simulink model "rocket_sim"  (R2023a)
settings: Solver=VariableStepAuto  StartTime=0.0  StopTime=480  RelTol=1e-3
undefined symbols (not defined in the file or in its folder): Earth, WGS84
libraries: simulink x55, slpidlib x10, aerolibconvert2 x7, matrix_library x4, aerolibasang x3, aerolibtransform2 x2, aerolibatmos2 x2, shared6dof x1, sharedtransform x1
(part 3 of 3)

== system rocket_sim/栅格舵控制器/栅格舵/F01 ==
  Th : Inport
  F : Inport  Port=2
  Constant : Constant  Value=0
  Saturation : Saturate  UpperLimit=1  LowerLimit=0
  Step1 : Step  Time=200  SampleTime=0
  Step2 : Step  Time=480  SampleTime=0
  Switch2 : Switch  Criteria=u2 > Threshold  SaturateOnIntegerOverflow=off  InputSameDT=off
  Switch3 : Switch  Criteria=u2 > Threshold  SaturateOnIntegerOverflow=off  InputSameDT=off
  Switch4 : Switch  Criteria=u2 > Threshold  SaturateOnIntegerOverflow=off  InputSameDT=off
  故障 : Subsystem
  退化 : Subsystem
  Out1 : Outport
  wires:
  Step1/1 -> Switch4/3
  退化/1(Out1) -> Switch3/3, Switch2/1
  F/1 -> Switch4/2
  Switch3/1 -> Switch2/3
  故障/1(Out1) -> Switch3/1
  Step2/1 -> Switch2/2
  Switch4/1 -> Switch3/2
  Th/1 -> 故障/1(Th), 退化/1(Th)
  Constant/1 -> Switch4/1
  Switch2/1 -> Saturation/1
  Saturation/1 -> Out1/1

== system rocket_sim/栅格舵控制器/栅格舵/F02 ==
  F : Inport
  Constant1 : Constant  Value=0
  Gain : Gain  Gain=0
  Gain1 : Gain
  Step : Step  Time=0  SampleTime=0
  Step1 : Step  Time=100  SampleTime=0
  Step2 : Step  Time=200  SampleTime=0
  Switch2 : Switch  Criteria=u2 > Threshold  SaturateOnIntegerOverflow=off  InputSameDT=off
  Switch4 : Switch  Criteria=u2 > Threshold  SaturateOnIntegerOverflow=off  InputSameDT=off
  Switch5 : Switch  Criteria=u2 > Threshold  SaturateOnIntegerOverflow=off  InputSameDT=off
  out2 : Outport
  wires:
  Switch5/1 -> Switch4/2
  Switch4/1 -> Switch2/3
  Constant1/1 -> Switch5/1
  Step1/1 -> Switch5/3
  Gain/1 -> Switch4/1
  Step2/1 -> Switch2/2
  Gain1/1 -> Switch4/3, Switch2/1
  Switch2/1 -> out2/1
  Step/1 -> Gain/1, Gain1/1
  F/1 -> Switch5/2

== system rocket_sim/栅格舵控制器/栅格舵/F03 ==
  Th : Inport
  F : Inport  Port=2
  Constant : Constant  Value=0
  Saturation : Saturate  UpperLimit=1  LowerLimit=0
  Step1 : Step  Time=200  SampleTime=0
  Step2 : Step  Time=480  SampleTime=0
  Switch2 : Switch  Criteria=u2 > Threshold  SaturateOnIntegerOverflow=off  InputSameDT=off
  Switch3 : Switch  Criteria=u2 > Threshold  SaturateOnIntegerOverflow=off  InputSameDT=off
  Switch4 : Switch  Criteria=u2 > Threshold  SaturateOnIntegerOverflow=off  InputSameDT=off
  故障 : Subsystem
  退化 : Subsystem
  Out1 : Outport
  wires:
  Step1/1 -> Switch4/3
  退化/1(Out1) -> Switch3/3, Switch2/1
  F/1 -> Switch4/2
  Switch3/1 -> Switch2/3
  故障/1(Out1) -> Switch3/1
  Step2/1 -> Switch2/2
  Switch4/1 -> Switch3/2
  Th/1 -> 故障/1(Th), 退化/1(Th)
  Switch2/1 -> Saturation/1
  Saturation/1 -> Out1/1
  Constant/1 -> Switch4/1

== system rocket_sim/栅格舵控制器/栅格舵/F04 ==
  F : Inport
  Constant1 : Constant  Value=0
  Gain : Gain  Gain=0
  Gain1 : Gain
  Step : Step  Time=0  SampleTime=0
  Step1 : Step  Time=100  SampleTime=0
  Step2 : Step  Time=200  SampleTime=0
  Switch2 : Switch  Criteria=u2 > Threshold  SaturateOnIntegerOverflow=off  InputSameDT=off
  Switch4 : Switch  Criteria=u2 > Threshold  SaturateOnIntegerOverflow=off  InputSameDT=off
  Switch5 : Switch  Criteria=u2 > Threshold  SaturateOnIntegerOverflow=off  InputSameDT=off
  out2 : Outport
  wires:
  Switch5/1 -> Switch4/2
  Switch4/1 -> Switch2/3
  Constant1/1 -> Switch5/1
  Step1/1 -> Switch5/3
  Gain/1 -> Switch4/1
  Step2/1 -> Switch2/2
  Gain1/1 -> Switch4/3, Switch2/1
  Switch2/1 -> out2/1
  Step/1 -> Gain/1, Gain1/1
  F/1 -> Switch5/2

== system rocket_sim/动力系统模块/喷管/F01/故障 ==
  Th : Inport
  Band-Limited White Noise1 : simulink/Sources/Band-Limited White Noise  Cov=[0.1]  Ts=0.1  seed=[23341]
  Clock1 : Clock
  Gain : Gain  Gain=0.9
  Gain2 : Gain  Gain=0.001
  Gain3 : Gain  Gain=-2.1950e-06
  Integrator1 : Integrator
  Math Function1 : Math
  Saturation : Saturate  UpperLimit=0.9  LowerLimit=0.5
  Sum2 : Sum  Inputs=|++
  Sum3 : Sum  Inputs=|++
  Out1 : Outport
  wires:
  Gain2/1 -> Sum2/2
  Th/1 -> Sum3/2
  Band-Limited White Noise1/1 -> Integrator1/1
  Clock1/1 -> Sum3/1
  Integrator1/1 -> Gain2/1
  Sum3/1 -> Gain3/1
  Gain3/1 -> Math Function1/1
  Saturation/1 -> Out1/1
  Sum2/1 -> Saturation/1
  Math Function1/1 -> Gain/1
  Gain/1 -> Sum2/1

== system rocket_sim/动力系统模块/喷管/F01/退化 ==
  Th : Inport
  Band-Limited White Noise1 : simulink/Sources/Band-Limited White Noise  Cov=[0.1]  Ts=0.1  seed=[23341]
  Clock1 : Clock
  Gain2 : Gain  Gain=0.0001
  Gain3 : Gain  Gain=-2.1950e-05
  Integrator1 : Integrator
  Math Function1 : Math
  Saturation : Saturate  UpperLimit=1  LowerLimit=0.5
  Scope : Scope
  Sum2 : Sum  Inputs=|++
  Sum3 : Sum  Inputs=|++
  Out1 : Outport
  wires:
  Gain2/1 -> Sum2/2
  Th/1 -> Sum3/2
  Band-Limited White Noise1/1 -> Integrator1/1
  Clock1/1 -> Sum3/1
  Integrator1/1 -> Gain2/1
  Sum3/1 -> Gain3/1
  Math Function1/1 -> Sum2/1
  Gain3/1 -> Math Function1/1
  Saturation/1 -> Out1/1
  Sum2/1 -> Scope/1, Saturation/1

== system rocket_sim/动力系统模块/氧涡轮/F01/故障 ==
  Th : Inport
  Band-Limited White Noise : simulink/Sources/Band-Limited White Noise  Cov=[0.1]  Ts=1  seed=[23341]
  Clock1 : Clock
  Gain : Gain  Gain=-4.65e-6
  Gain1 : Gain  Gain=0.8
  Integrator : Integrator
  Math Function : Math
  Saturation : Saturate  UpperLimit=1  LowerLimit=0.5
  Sum : Sum  Inputs=|++
  Sum1 : Sum  Inputs=|++
  σ : Gain  Gain=1e-3
  Out1 : Outport
  wires:
  Band-Limited White Noise/1 -> Integrator/1
  Clock1/1 -> Sum/1
  Integrator/1 -> σ/1
  Gain/1 -> Math Function/1
  σ/1 -> Sum1/2
  Sum/1 -> Gain/1
  Sum1/1 -> Saturation/1
  Saturation/1 -> Out1/1
  Math Function/1 -> Gain1/1
  Gain1/1 -> Sum1/1
  Th/1 -> Sum/2

== system rocket_sim/动力系统模块/氧涡轮/F01/退化 ==
  Th : Inport
  Band-Limited White Noise : simulink/Sources/Band-Limited White Noise  Cov=[0.1]  Ts=1  seed=[23341]
  Clock1 : Clock
  Gain : Gain  Gain=-4.65e-5
  Integrator : Integrator
  Math Function : Math
  Saturation : Saturate  UpperLimit=1  LowerLimit=0.5
  Sum : Sum  Inputs=|++
  Sum1 : Sum  Inputs=|++
  σ : Gain  Gain=1e-3
  Out1 : Outport
  wires:
  Band-Limited White Noise/1 -> Integrator/1
  Th/1 -> Sum/2
  Clock1/1 -> Sum/1
  Integrator/1 -> σ/1
  Gain/1 -> Math Function/1
  Math Function/1 -> Sum1/1
  σ/1 -> Sum1/2
  Sum/1 -> Gain/1
  Sum1/1 -> Saturation/1
  Saturation/1 -> Out1/1

== system rocket_sim/动力系统模块/液氧主阀/F01/故障 ==
  Th : Inport
  Band-Limited White Noise : simulink/Sources/Band-Limited White Noise  Cov=[0.1]  Ts=0.1  seed=[23341]
  Clock2 : Clock
  Constant : Constant  Value=0.9
  Gain : Gain  Gain=-0.00012
  Gain1 : Gain  Gain=0.0001
  Integrator : Integrator
  MATLAB Function1 : MATLAB Function  TreatAsAtomicUnit=on
  Sum : Sum  Inputs=|++
  Sum1 : Sum  Inputs=|+++
  Out1 : Outport
  wires:
  Gain/1 -> Sum1/1
  Th/1 -> Sum/2
  MATLAB Function1/1(y) -> Gain/1
  Sum/1 -> MATLAB Function1/1(t)
  Constant/1 -> Sum1/2
  Clock2/1 -> Sum/1
  Sum1/1 -> Out1/1
  Gain1/1 -> Sum1/3
  Band-Limited White Noise/1 -> Integrator/1
  Integrator/1 -> Gain1/1

== system rocket_sim/动力系统模块/液氧主阀/F01/退化 ==
  Th : Inport
  Band-Limited White Noise : simulink/Sources/Band-Limited White Noise  Cov=[0.1]  Ts=0.1  seed=[23341]
  Clock2 : Clock
  Constant : Constant
  Gain : Gain  Gain=-0.0012
  Gain1 : Gain  Gain=0.0001
  Integrator : Integrator
  MATLAB Function1 : MATLAB Function  TreatAsAtomicUnit=on
  Sum : Sum  Inputs=|++
  Sum1 : Sum  Inputs=|+++
  Out1 : Outport
  wires:
  Gain/1 -> Sum1/1
  Th/1 -> Sum/2
  MATLAB Function1/1(y) -> Gain/1
  Sum/1 -> MATLAB Function1/1(t)
  Constant/1 -> Sum1/2
  Clock2/1 -> Sum/1
  Sum1/1 -> Out1/1
  Band-Limited White Noise/1 -> Integrator/1
  Integrator/1 -> Gain1/1
  Gain1/1 -> Sum1/3

== system rocket_sim/动力系统模块/液氧泵/F01/故障 ==
  Th : Inport
  Add1 : Sum  Inputs=+++
  Band-Limited White Noise1 : simulink/Sources/Band-Limited White Noise  Cov=[0.1]  Ts=1  seed=[23341]
  Clock1 : Clock
  Constant3 : Constant  Value=0.8
  Integrator1 : Integrator
  Scope : Scope
  Sum : Sum  Inputs=|++
  μ1 : Gain  Gain=-4.1667e-06
  σ1 : Gain  Gain=1e-3
  Out1 : Outport
  wires:
  Th/1 -> Sum/2
  Sum/1 -> Scope/1, μ1/1
  Clock1/1 -> Sum/1
  Band-Limited White Noise1/1 -> Integrator1/1
  Integrator1/1 -> σ1/1
  σ1/1 -> Add1/2
  μ1/1 -> Add1/3
  Constant3/1 -> Add1/1
  Add1/1 -> Out1/1

== system rocket_sim/动力系统模块/液氧泵/F01/退化 ==
  Th : Inport
  Add : Sum  Inputs=+++
  Band-Limited White Noise : simulink/Sources/Band-Limited White Noise  Cov=[0.1]  Ts=1  seed=[23341]
  Clock : Clock
  Constant2 : Constant
  Integrator : Integrator
  Sum : Sum  Inputs=|++
  μ : Gain  Gain=-6.94e-5
  σ : Gain  Gain=1e-3
  Out1 : Outport
  wires:
  Band-Limited White Noise/1 -> Integrator/1
  σ/1 -> Add/2
  Integrator/1 -> σ/1
  Constant2/1 -> Add/1
  Add/1 -> Out1/1
  μ/1 -> Add/3
  Clock/1 -> Sum/1
  Sum/1 -> μ/1
  Th/1 -> Sum/2

== system rocket_sim/动力系统模块/液氧管路/F01/故障 ==
  Th : Inport
  Add1 : Sum  Inputs=+++
  Band-Limited White Noise1 : simulink/Sources/Band-Limited White Noise  Cov=[0.1]  Ts=1  seed=[23341]
  Clock1 : Clock
  Constant3 : Constant  Value=0.8
  Integrator1 : Integrator
  Scope : Scope
  Sum : Sum  Inputs=|++
  μ1 : Gain  Gain=-2.0833e-06
  σ1 : Gain  Gain=1e-3
  Out1 : Outport
  wires:
  Th/1 -> Sum/2
  Sum/1 -> Scope/1, μ1/1
  Clock1/1 -> Sum/1
  Band-Limited White Noise1/1 -> Integrator1/1
  Integrator1/1 -> σ1/1
  σ1/1 -> Add1/2
  μ1/1 -> Add1/3
  Constant3/1 -> Add1/1
  Add1/1 -> Out1/1

== system rocket_sim/动力系统模块/液氧管路/F01/退化 ==
  Th : Inport
  Add : Sum  Inputs=+++
  Band-Limited White Noise : simulink/Sources/Band-Limited White Noise  Cov=[0.1]  Ts=1  seed=[23341]
  Clock : Clock
  Constant2 : Constant
  Integrator : Integrator
  Sum : Sum  Inputs=|++
  μ : Gain  Gain=-2.0833e-05
  σ : Gain  Gain=1e-3
  Out1 : Outport
  wires:
  Band-Limited White Noise/1 -> Integrator/1
  σ/1 -> Add/2
  Integrator/1 -> σ/1
  Constant2/1 -> Add/1
  Add/1 -> Out1/1
  μ/1 -> Add/3
  Clock/1 -> Sum/1
  Sum/1 -> μ/1
  Th/1 -> Sum/2

== system rocket_sim/动力系统模块/煤油主阀/F01/故障 ==
  Th : Inport
  Band-Limited White Noise : simulink/Sources/Band-Limited White Noise  Cov=[0.1]  Ts=0.1  seed=[23341]
  Clock2 : Clock
  Constant : Constant  Value=0.9
  Gain : Gain  Gain=-0.00012
  Gain1 : Gain  Gain=0.0001
  Integrator : Integrator
  MATLAB Function1 : MATLAB Function  TreatAsAtomicUnit=on
  Sum : Sum  Inputs=|++
  Sum1 : Sum  Inputs=|+++
  Out1 : Outport
  wires:
  Gain/1 -> Sum1/1
  Th/1 -> Sum/2
  MATLAB Function1/1(y) -> Gain/1
  Sum/1 -> MATLAB Function1/1(t)
  Constant/1 -> Sum1/2
  Clock2/1 -> Sum/1
  Sum1/1 -> Out1/1
  Gain1/1 -> Sum1/3
  Band-Limited White Noise/1 -> Integrator/1
  Integrator/1 -> Gain1/1

== system rocket_sim/动力系统模块/煤油主阀/F01/退化 ==
  Th : Inport
  Band-Limited White Noise : simulink/Sources/Band-Limited White Noise  Cov=[0.1]  Ts=0.1  seed=[23341]
  Clock2 : Clock
  Constant : Constant
  Gain : Gain  Gain=-0.0012
  Gain1 : Gain  Gain=0.0001
  Integrator : Integrator
  MATLAB Function1 : MATLAB Function  TreatAsAtomicUnit=on
  Sum : Sum  Inputs=|++
  Sum1 : Sum  Inputs=|+++
  Out1 : Outport
  wires:
  Gain/1 -> Sum1/1
  Th/1 -> Sum/2
  MATLAB Function1/1(y) -> Gain/1
  Sum/1 -> MATLAB Function1/1(t)
  Constant/1 -> Sum1/2
  Clock2/1 -> Sum/1
  Sum1/1 -> Out1/1
  Band-Limited White Noise/1 -> Integrator/1
  Integrator/1 -> Gain1/1
  Gain1/1 -> Sum1/3

== system rocket_sim/动力系统模块/煤油泵/F01/故障 ==
  Th : Inport
  Add1 : Sum  Inputs=+++
  Band-Limited White Noise1 : simulink/Sources/Band-Limited White Noise  Cov=[0.1]  Ts=1  seed=[23341]
  Clock1 : Clock
  Constant3 : Constant  Value=0.8
  Integrator1 : Integrator
  Scope : Scope
  Sum : Sum  Inputs=|++
  μ1 : Gain  Gain=-4.1667e-06
  σ1 : Gain  Gain=1e-3
  Out1 : Outport
  wires:
  Th/1 -> Sum/2
  Sum/1 -> Scope/1, μ1/1
  Clock1/1 -> Sum/1
  Band-Limited White Noise1/1 -> Integrator1/1
  Integrator1/1 -> σ1/1
  σ1/1 -> Add1/2
  μ1/1 -> Add1/3
  Constant3/1 -> Add1/1
  Add1/1 -> Out1/1

== system rocket_sim/动力系统模块/煤油泵/F01/退化 ==
  Th : Inport
  Add : Sum  Inputs=+++
  Band-Limited White Noise : simulink/Sources/Band-Limited White Noise  Cov=[0.1]  Ts=1  seed=[23341]
  Clock : Clock
  Constant2 : Constant
  Integrator : Integrator
  Sum : Sum  Inputs=|++
  μ : Gain  Gain=-6.94e-5
  σ : Gain  Gain=1e-3
  Out1 : Outport
  wires:
  Band-Limited White Noise/1 -> Integrator/1
  σ/1 -> Add/2
  Integrator/1 -> σ/1
  Constant2/1 -> Add/1
  Add/1 -> Out1/1
  μ/1 -> Add/3
  Clock/1 -> Sum/1
  Sum/1 -> μ/1
  Th/1 -> Sum/2

== system rocket_sim/动力系统模块/煤油涡轮/F01/故障 ==
  Th : Inport
  Band-Limited White Noise : simulink/Sources/Band-Limited White Noise  Cov=[0.1]  Ts=1  seed=[23341]
  Clock1 : Clock
  Gain : Gain  Gain=-4.65e-5
  Gain1 : Gain  Gain=0.8
  Integrator : Integrator
  Math Function : Math
  Saturation : Saturate  UpperLimit=1  LowerLimit=0.5
  Sum : Sum  Inputs=|++
  Sum1 : Sum  Inputs=|++
  σ : Gain  Gain=1e-3
  Out1 : Outport
  wires:
  Band-Limited White Noise/1 -> Integrator/1
  Clock1/1 -> Sum/1
  Integrator/1 -> σ/1
  Gain/1 -> Math Function/1
  σ/1 -> Sum1/2
  Sum/1 -> Gain/1
  Sum1/1 -> Saturation/1
  Saturation/1 -> Out1/1
  Math Function/1 -> Gain1/1
  Gain1/1 -> Sum1/1
  Th/1 -> Sum/2

== system rocket_sim/动力系统模块/煤油涡轮/F01/退化 ==
  Th : Inport
  Band-Limited White Noise : simulink/Sources/Band-Limited White Noise  Cov=[0.1]  Ts=1  seed=[23341]
  Clock1 : Clock
  Gain : Gain  Gain=-4.65e-5
  Integrator : Integrator
  Math Function : Math
  Saturation : Saturate  UpperLimit=1  LowerLimit=0.5
  Sum : Sum  Inputs=|++
  Sum1 : Sum  Inputs=|++
  σ : Gain  Gain=1e-3
  Out1 : Outport
  wires:
  Band-Limited White Noise/1 -> Integrator/1
  Th/1 -> Sum/2
  Clock1/1 -> Sum/1
  Integrator/1 -> σ/1
  Gain/1 -> Math Function/1
  Math Function/1 -> Sum1/1
  σ/1 -> Sum1/2
  Sum/1 -> Gain/1
  Sum1/1 -> Saturation/1
  Saturation/1 -> Out1/1

== system rocket_sim/动力系统模块/煤油管路/F01/故障 ==
  Th : Inport
  Add1 : Sum  Inputs=+++
  Band-Limited White Noise1 : simulink/Sources/Band-Limited White Noise  Cov=[0.1]  Ts=1  seed=[23341]
  Clock1 : Clock
  Constant3 : Constant  Value=0.8
  Integrator1 : Integrator
  Scope : Scope
  Sum : Sum  Inputs=|++
  μ1 : Gain  Gain=-2.0833e-06
  σ1 : Gain  Gain=1e-3
  Out1 : Outport
  wires:
  Th/1 -> Sum/2
  Sum/1 -> Scope/1, μ1/1
  Clock1/1 -> Sum/1
  Band-Limited White Noise1/1 -> Integrator1/1
  Integrator1/1 -> σ1/1
  σ1/1 -> Add1/2
  μ1/1 -> Add1/3
  Constant3/1 -> Add1/1
  Add1/1 -> Out1/1

== system rocket_sim/动力系统模块/煤油管路/F01/退化 ==
  Th : Inport
  Add : Sum  Inputs=+++
  Band-Limited White Noise : simulink/Sources/Band-Limited White Noise  Cov=[0.1]  Ts=1  seed=[23341]
  Clock : Clock
  Constant2 : Constant
  Integrator : Integrator
  Sum : Sum  Inputs=|++
  μ : Gain  Gain=-2.0833e-05
  σ : Gain  Gain=1e-3
  Out1 : Outport
  wires:
  Band-Limited White Noise/1 -> Integrator/1
  σ/1 -> Add/2
  Integrator/1 -> σ/1
  Constant2/1 -> Add/1
  Add/1 -> Out1/1
  μ/1 -> Add/3
  Clock/1 -> Sum/1
  Sum/1 -> μ/1
  Th/1 -> Sum/2

== system rocket_sim/动力系统模块/燃气发生器/F01/故障 ==
  Th : Inport
  Band-Limited White Noise : simulink/Sources/Band-Limited White Noise  Cov=[0.1]  Ts=0.1  seed=[23341]
  Clock : Clock
  Constant1 : Constant
  Gain : Gain  Gain=-2.1950e-05
  Gain1 : Gain  Gain=0.001
  Gain2 : Gain  Gain=0.9
  Integrator : Integrator
  Math Function : Math
  Saturation : Saturate  LowerLimit=0
  Sum : Sum  Inputs=|--+
  Sum1 : Sum  Inputs=|++
  Fg2 : Outport
  wires:
  Constant1/1 -> Sum/3
  Gain1/1 -> Sum/2
  Gain/1 -> Math Function/1
  Band-Limited White Noise/1 -> Integrator/1
  Integrator/1 -> Gain1/1
  Clock/1 -> Sum1/1
  Th/1 -> Sum1/2
  Sum1/1 -> Gain/1
  Math Function/1 -> Gain2/1
  Gain2/1 -> Sum/1
  Sum/1 -> Saturation/1
  Saturation/1 -> Fg2/1

== system rocket_sim/动力系统模块/燃气发生器/F01/退化 ==
  Th : Inport
  Band-Limited White Noise : simulink/Sources/Band-Limited White Noise  Cov=[0.1]  Ts=0.1  seed=[23341]
  Clock : Clock
  Constant1 : Constant
  Gain : Gain  Gain=-2.1950e-05
  Gain1 : Gain  Gain=0.001
  Integrator : Integrator
  Math Function : Math
  Saturation : Saturate  LowerLimit=0
  Scope : Scope
  Sum : Sum  Inputs=|-++
  Sum1 : Sum  Inputs=|++
  Fg2 : Outport
  wires:
  Math Function/1 -> Scope/1, Sum/1
  Constant1/1 -> Sum/3
  Gain1/1 -> Sum/2
  Gain/1 -> Math Function/1
  Band-Limited White Noise/1 -> Integrator/1
  Integrator/1 -> Gain1/1
  Clock/1 -> Sum1/1
  Th/1 -> Sum1/2
  Sum1/1 -> Gain/1
  Sum/1 -> Saturation/1
  Saturation/1 -> Fg2/1

== system rocket_sim/动力系统模块/燃烧室/F01/故障 ==
  Th : Inport
  Add1 : Sum  Inputs=+++
  Band-Limited White Noise1 : simulink/Sources/Band-Limited White Noise  Cov=[0.1]  Ts=0.1  seed=[23341]
  Clock1 : Clock
  Constant2 : Constant  Value=1.2
  Constant3 : Constant
  Gain2 : Gain  Gain=0.0001
  Gain3 : Gain  Gain=-2.1950e-05
  Integrator1 : Integrator
  Math Function1 : Math
  Saturation : Saturate  UpperLimit=1.5  LowerLimit=1
  Sum2 : Sum  Inputs=|-+
  Sum3 : Sum  Inputs=|++
  Out1 : Outport
  wires:
  Sum3/1 -> Gain3/1
  Th/1 -> Sum3/2
  Band-Limited White Noise1/1 -> Integrator1/1
  Integrator1/1 -> Gain2/1
  Constant2/1 -> Add1/1
  Gain2/1 -> Add1/2
  Gain3/1 -> Math Function1/1
  Sum2/1 -> Add1/3
  Math Function1/1 -> Sum2/1
  Clock1/1 -> Sum3/1
  Constant3/1 -> Sum2/2
  Add1/1 -> Saturation/1
  Saturation/1 -> Out1/1

== system rocket_sim/动力系统模块/燃烧室/F01/退化 ==
  Th : Inport
  Add : Sum  Inputs=+++
  Band-Limited White Noise : simulink/Sources/Band-Limited White Noise  Cov=[0.1]  Ts=0.1  seed=[23341]
  Clock : Clock
  Constant : Constant
  Constant1 : Constant
  Gain : Gain  Gain=0.001
  Gain1 : Gain  Gain=-2.1950e-05
  Integrator : Integrator
  Math Function : Math
  Saturation : Saturate  UpperLimit=1.5  LowerLimit=1
  Scope : Scope
  Scope1 : Scope
  Sum : Sum  Inputs=|-+
  Sum1 : Sum  Inputs=|++
  Out1 : Outport
  wires:
  Integrator/1 -> Gain/1
  Math Function/1 -> Scope1/1, Sum/1
  Gain/1 -> Add/2
  Th/1 -> Sum1/2
  Constant/1 -> Add/1
  Band-Limited White Noise/1 -> Integrator/1
  Gain1/1 -> Math Function/1
  Sum1/1 -> Gain1/1
  Clock/1 -> Sum1/1
  Sum/1 -> Scope/1, Add/3
  Constant1/1 -> Sum/2
  Add/1 -> Saturation/1
  Saturation/1 -> Out1/1

== system rocket_sim/姿态推进器/RCS/F01/故障 ==
  Th : Inport
  Band-Limited White Noise : simulink/Sources/Band-Limited White Noise  Cov=[0.1]  Ts=0.1  seed=[23341]
  Clock : Clock
  Constant4 : Constant  Value=0.8
  Gain1 : Gain  Gain=-4e-05
  Gain3 : Gain  Gain=0.001
  Integrator : Integrator
  Saturation1 : Saturate  UpperLimit=1  LowerLimit=0
  Sum : Sum  Inputs=|+++
  Sum1 : Sum  Inputs=|++
  Out1 : Outport
  wires:
  Band-Limited White Noise/1 -> Integrator/1
  Th/1 -> Sum1/2
  Constant4/1 -> Sum/3
  Integrator/1 -> Gain3/1
  Gain3/1 -> Sum/2
  Sum/1 -> Saturation1/1
  Clock/1 -> Sum1/1
  Sum1/1 -> Gain1/1
  Gain1/1 -> Sum/1
  Saturation1/1 -> Out1/1

== system rocket_sim/姿态推进器/RCS/F01/退化 ==
  Th : Inport
  Band-Limited White Noise : simulink/Sources/Band-Limited White Noise  Cov=[0.1]  Ts=0.1  seed=[23341]
  Clock : Clock
  Constant4 : Constant
  Gain1 : Gain  Gain=-4e-05
  Gain3 : Gain  Gain=0.001
  Integrator : Integrator
  Saturation1 : Saturate  UpperLimit=1  LowerLimit=0
  Sum : Sum  Inputs=|+++
  Sum1 : Sum  Inputs=|++
  Out1 : Outport
  wires:
  Band-Limited White Noise/1 -> Integrator/1
  Th/1 -> Sum1/2
  Constant4/1 -> Sum/3
  Integrator/1 -> Gain3/1
  Gain3/1 -> Sum/2
  Sum/1 -> Saturation1/1
  Clock/1 -> Sum1/1
  Sum1/1 -> Gain1/1
  Gain1/1 -> Sum/1
  Saturation1/1 -> Out1/1

== system rocket_sim/栅格舵控制器/栅格舵/F01/故障 ==
  Th : Inport
  Band-Limited White Noise : simulink/Sources/Band-Limited White Noise  Cov=[0.1]  Ts=0.1  seed=[23341]
  Clock2 : Clock
  Constant : Constant  Value=0.8
  Gain3 : Gain  Gain=-4e-05
  Gain4 : Gain  Gain=0.001
  Integrator : Integrator
  Sum2 : Sum  Inputs=|++
  Sum3 : Sum  Inputs=|+++
  Out1 : Outport
  wires:
  Sum2/1 -> Gain3/1
  Gain3/1 -> Sum3/1
  Sum3/1 -> Out1/1
  Constant/1 -> Sum3/3
  Clock2/1 -> Sum2/1
  Th/1 -> Sum2/2
  Integrator/1 -> Gain4/1
  Gain4/1 -> Sum3/2
  Band-Limited White Noise/1 -> Integrator/1

== system rocket_sim/栅格舵控制器/栅格舵/F01/退化 ==
  Th : Inport
  Band-Limited White Noise : simulink/Sources/Band-Limited White Noise  Cov=[0.1]  Ts=0.1  seed=[23341]
  Clock2 : Clock
  Constant : Constant
  Gain3 : Gain  Gain=-4e-05
  Gain4 : Gain  Gain=0.001
  Integrator : Integrator
  Sum2 : Sum  Inputs=|++
  Sum3 : Sum  Inputs=|+++
  Out1 : Outport
  wires:
  Sum2/1 -> Gain3/1
  Gain3/1 -> Sum3/1
  Sum3/1 -> Out1/1
  Constant/1 -> Sum3/3
  Clock2/1 -> Sum2/1
  Th/1 -> Sum2/2
  Integrator/1 -> Gain4/1
  Gain4/1 -> Sum3/2
  Band-Limited White Noise/1 -> Integrator/1

== system rocket_sim/栅格舵控制器/栅格舵/F03/故障 ==
  Th : Inport
  Band-Limited White Noise : simulink/Sources/Band-Limited White Noise  Cov=[0.1]  Ts=0.1  seed=[23341]
  Clock2 : Clock
  Constant : Constant  Value=0.2
  Gain3 : Gain  Gain=0
  Gain4 : Gain  Gain=0.001
  Integrator : Integrator
  Sum2 : Sum  Inputs=|++
  Sum3 : Sum  Inputs=|+++
  Out1 : Outport
  wires:
  Sum2/1 -> Gain3/1
  Gain3/1 -> Sum3/1
  Sum3/1 -> Out1/1
  Constant/1 -> Sum3/3
  Clock2/1 -> Sum2/1
  Th/1 -> Sum2/2
  Integrator/1 -> Gain4/1
  Gain4/1 -> Sum3/2
  Band-Limited White Noise/1 -> Integrator/1

== system rocket_sim/栅格舵控制器/栅格舵/F03/退化 ==
  Th : Inport
  Band-Limited White Noise : simulink/Sources/Band-Limited White Noise  Cov=[0.1]  Ts=0.1  seed=[23341]
  Clock2 : Clock
  Constant : Constant  Value=0
  Gain3 : Gain  Gain=4e-05
  Gain4 : Gain  Gain=0.001
  Integrator : Integrator
  Sum2 : Sum  Inputs=|++
  Sum3 : Sum  Inputs=|+++
  Out1 : Outport
  wires:
  Sum2/1 -> Gain3/1
  Gain3/1 -> Sum3/1
  Sum3/1 -> Out1/1
  Constant/1 -> Sum3/3
  Clock2/1 -> Sum2/1
  Th/1 -> Sum2/2
  Integrator/1 -> Gain4/1
  Gain4/1 -> Sum3/2
  Band-Limited White Noise/1 -> Integrator/1

== matlab function rocket_sim/动力系统模块/液氧管路/MATLAB Function ==
  data: P_i input; dm_o output; dm_i input; m input; Fl1 input; P_e output; Fl2 input
function [dm_o, P_e] = pipe_dynamics(P_i,  dm_i,m, Fl1, Fl2)
    % 参数设置
    L = 0;    % 惯性流阻系数
    K = 0;    % 管路流阻系数
    C = 1;  % 流容系数
    f = 0.02;
    D = 0.9;
   LL = 10;
    A = (D/2)^2/4;
    rho = 820;
    delta_P = f*LL/(2*rho*1141*A*A*D)*dm_i^2;
  


    dm_o = dm_i*Fl1;

    P_e = (P_i -  L*dm_o/Fl1 - Fl2*K*m^2-delta_P)/C;

    
end

== matlab function rocket_sim/动力系统模块/煤油主阀/MATLAB Function ==
  data: Pi input; Pe output; dmi input; Fv1 input; dmo output
function [Pe,dmo] = fcn(Pi,dmi,Fv1)

uF = 0.8;
rho = 820;
Pe = Pi - (dmi/uF)^2/(2*rho)/2.5;
dmo = Fv1*dmi;

== matlab function rocket_sim/动力系统模块/煤油主阀/F01/退化/MATLAB Function1 ==
  data: t input; y output
function y = fcn(t)

y = t^0.5;

== matlab function rocket_sim/动力系统模块/煤油主阀/F01/故障/MATLAB Function1 ==
  data: t input; y output
function y = fcn(t)

y = t^0.5;

== matlab function rocket_sim/动力系统模块/液氧主阀/F01/故障/MATLAB Function1 ==
  data: t input; y output
function y = fcn(t)

y = t^0.5;

== matlab function rocket_sim/动力系统模块/液氧主阀/F01/退化/MATLAB Function1 ==
  data: t input; y output
function y = fcn(t)

y = t^0.5;

== matlab function rocket_sim/动力系统模块/液氧主阀/MATLAB Function ==
  data: Pi input; Pe output; dmi input; Fv1 input; dmo output
function [Pe,dmo] = fcn(Pi,dmi,Fv1)

uF = 0.8;
rho = 1141;
Pe = Pi - (dmi/uF)^2/(2*rho)/5;
dmo = Fv1*dmi;

== matlab function rocket_sim/动力系统模块/燃气发生器/燃气发生器 ==
  data: dmo input; gamma output; RT output; dmf input; dmg input; Pe input; dme output; P output; Fg1 input; Fg2 input
function [gamma, RT,dme, P] = Gas_generator(dmo,dmf,dmg,Pe,Fg1,Fg2)

RT = 9e6;
gamma = 1.3;
dme = 6.19/2;

dm = dmo + dmf + dmg -(1+Fg2)*dme;

V = 0.05;
dP = dm*RT/V;
zeta = 1;
A = 1;
xishu1 = sqrt(gamma*(2/(gamma+1))^((gamma+1)/(gamma-1)));
xishu2 = sqrt(RT)/(zeta*A*Fg1);
P =(dme*xishu2/xishu1 + dP - Pe)*30/(1e10);

== matlab function rocket_sim/动力系统模块/燃烧室/燃烧室 ==
  data: dmo input; Pe output; dmf input; dmg input; dm output; Fr1 input
function [Pe,dm] = chamber(dmo,dmf,dmg,Fr1)

dm = dmo + dmf + dmg;

R = 400;
T = 3500;
gamma = 1.3;
r1 = sqrt(gamma*(2/(gamma+1))^((gamma+1)/(gamma-1)));
r2 = sqrt(R*T)/50;
A = 0.0205;

Pe = (dm/(r1*A*Fr1))*r2;

== matlab function rocket_sim/动力系统模块/喷管/喷管 ==
  data: dm input; F output; P0 input; Pi input; ve output; Fwg1 input
function [F,ve] = chamber(dm,P0,Pi,Fwg1)

A = 0.205;
R = 300;
T = 3300;
gamma = 1.3;
k = (gamma-1)/gamma;
eta = 0.85;
L = 0.99;
ve = sqrt(gamma*2/(gamma-1) * R * T*L^k)*Fwg1;
F = (dm * ve + (Pi - P0)*A)*eta;

== matlab function rocket_sim/空气动力学模块/MATLAB Function ==
  data: rho input; F_a output; V input; M_a output; deltaAC input; deltaBD input; q output
function [F_a, M_a,q] = aero_force_moment(rho, V,deltaAC,deltaBD)
% aero_force_moment 计算气动力和气动力矩（三维体轴系下）
%
% 输入参数：
%   rho  - 空气密度 (kg/m^3)
%   V    - 相对气流速度 (m/s)
%   S    - 参考面积 (m^2)
%   l    - 参考长度 (m)
%   C_D  - 阻力系数（沿 -X 轴）
%   C_Y  - 侧力系数（沿 Y 轴）
%   C_L  - 升力系数（沿 -Z 轴）
%   C_l  - 滚转力矩系数（绕 X 轴）
%   C_m  - 俯仰力矩系数（绕 Y 轴）
%   C_n  - 偏航力矩系数（绕 Z 轴）
%
% 输出参数：
%   F_a  - 3×1 气动力向量 [N]
%   M_a  - 3×1 气动力矩向量 [N·m]
S = 10.52;            % m^2
l = 1.83;            % m

C_D = 0.3;
C_Y = 0.05;
C_L = 0.2;

C_l = 0.00001;
C_m = 0.1;
C_n = 0.01;

q = 0.5 * rho * V^2;  % 动压

% 气动力向量（在体轴系下：X-头部，Y-右，Z-下）
F_a = q * S * [-C_D; C_Y; -C_L];

    % 气动力矩向量
M_a = q * S * l * [2*C_l; C_m*deltaAC; 2*C_n*deltaBD];
%M_a = 0;
end

== matlab function rocket_sim/动力系统模块/液氧泵/液氧泵 ==
  data: Pi input; Pe output; dm input; n input; Np output; Fp1 input
function [Pe, Np] = oxygen_pump(Pi, dm, n, Fp1)
%泵扬程经验系数
up1 = -3.77981754e-10;
up2 = 1.12865599e-07;
up3 = 2.12375184e-04;

Pe = (up1*n^2 + up2*n*dm + up3*dm^2)*Fp1 + Pi;

%功率经验系数

vn1 = 9.70418259e-11;
vn2 = -4.15546957e-08;
vn3 = 5.76242575e-06;

Np = vn1*n^3 + vn2*n^2*dm + vn3*n*dm^2;

== matlab function rocket_sim/制导模块/MATLAB Function ==
  data: t input; theta output
function theta = pitch_angle(t)
%PITCH_ANGLE Computes pitch angle over time with smooth rise and fall
%   Input:
%       t - time in seconds (can be scalar or vector)
%   Output:
%       theta - pitch angle in degrees

    % 参数
    % 参数定义
    theta1 = 45;
    theta2 = 45;
    theta3 = 0;
    t1 = 140;    % 上升结束
    t2 = 155;    % 保持结束
    t3 = 330;    % 下降结束
    t4 = 480;

    % 初始化输出
    theta = zeros(size(t));

    for i = 1:length(t)
        ti = t(i);

        if ti <= t1
            % 上升阶段：0 → 45°（余弦缓变）
            theta(i) = theta1 * 0.5 * (1 - cos(pi * ti / t1));

        elseif ti <= t2
            % 保持阶段
            tau1 = (ti - t1) / (t2 - t1);  % 归一化时间 [0,1]
            theta(i) = theta1 + 0.5 * (1 - cos(pi * tau1)) * (theta2 - theta1);
        elseif ti <= t3
                theta(i) =  theta2;
        elseif ti <= t4
            % 下降阶段：45° → 0（余弦缓变）
            tau = (ti - t3) / (t4 - t3);  % 归一化时间 [0,1]
            theta(i) = theta2* 0.5 * (1 + cos(pi * tau));

        else
            % 超出480秒后保持为0°
            theta(i) = 0;
        end
    end
end

== matlab function rocket_sim/空气动力学模块1/MATLAB Function ==
  data: CD output; CY output; CL output; alpha input; beta input; delta_a input; delta_e input; Cl output; Cm output; Cn output; delta_r input; omega_x input; omega_y input; omega_z input; Ma input; V input
function [CD,CY,CL,Cl,Cm,Cn] = aeroCoeffs(alpha,beta,delta_a, delta_e, delta_r,omega_x,omega_y,omega_z, Ma, V)
% 气动系数
CL_0 = 0.6;
CL_alpha = 0.15;
CL_delE = 0.0;
CL_Ma = 0;

CL = CL_0 + CL_alpha*alpha + CL_delE*delta_e + CL_Ma*Ma;

CD_0 = 0.3;
CD_alpha = 0.025;
CD_delE = 0.0;
CD_Ma = 0;

CD = CD_0 + CD_alpha*alpha + CD_delE*delta_e + CD_Ma*Ma;

CY_beta = 0.05;
CY_delR = 0.0;
CY_delA = 0.0;
CY_omega_x = 0;
CY_omega_z = 0;
lL = 1.8;
lc = 3.66;

CY = CY_beta*beta + CY_delR*delta_r + CY_delA*delta_a + (CY_omega_x*omega_x + CY_omega_z*omega_z)*lL/(2*V);

Cl_beta = 0;
Cl_delA = 0.10;
Cl_delR = 0;
Cl_omega_x = 0;
Cl_omega_z = 0;

Cl = Cl_beta*beta + Cl_delA*delta_a + Cl_delR*delta_r + (Cl_omega_x*omega_x + Cl_omega_z*omega_z)*lL/(2*V);

Cm_0 = 0;
Cm_alpha = 0;
Cm_delE = 0.085;
Cm_alpha2 = 0;
Cm_omega_y = 0;

Cm = Cm_0 + Cm_alpha*alpha + Cm_delE*delta_e + (Cm_alpha2*alpha + Cm_omega_y*omega_y)*lc/(2*V);

Cn_beta = 0;
Cn_delR = 0.12;
Cn_delA = 0;
Cn_omega_x = 0;
Cn_omega_z = 0;

Cn = Cn_beta*beta + Cn_delR*delta_r + Cn_delA*delta_a + (Cn_omega_x*omega_x + Cn_omega_z*omega_z)*lL/(2*V);

== matlab function rocket_sim/动力系统模块/煤油泵/煤油泵 ==
  data: Pi input; Pe output; dm input; n input; Np output; Fp1 input
function [Pe, Np] = kerosene_pump(Pi, dm, n, Fp1)
%泵扬程经验系数
up1 = -6.36117673e-24;
up2 = 4.54933201e-21;
up3 = 1.33087861e-03;

Pe = (up1*n^2 + up2*n*dm + up3*dm^2)*Fp1 + Pi;

%功率经验系数

vn1 = 9.68405071e-11;
vn2 = -9.31262763e-08;
vn3 = 2.89994238e-05;

Np = vn1*n^3 + vn2*n^2*dm + vn3*n*dm^2;

== matlab function rocket_sim/动力系统模块/氧涡轮/氧涡轮 ==
  data: Pi input; Pe input; Np input; RTi input; gamma input; dm input; t input; Ftg1 input; Ftg2 input; Ftg3 input; n output; eta output
function [n,eta]  = fcn(Pi, Pe, Np, RTi, gamma, dm, t , Ftg1, Ftg2, Ftg3)
Np = Np*1000;
N = Np*(1+Ftg2)/Ftg1;
k =  gamma/(gamma - 1);
theta = 1;
P0 = Pi*(theta+(1-theta)*(Pe/Pi)^(1/k))^(k);
ve = sqrt(2*k*RTi*(1-(Pe/P0)^(1/k)));
eta = 2*N*dm*Ftg3/(ve^2);

b1 = -1;
b2 = 4;
b3 = -eta;

coeff = [b1, b2, b3];
x_roots = roots(coeff);

phi = max(x_roots(x_roots > 0));

n = real(ve * phi/0.666);

if t <=1
    n =35500;
end

== matlab function rocket_sim/动力系统模块/煤油涡轮/氧涡轮 ==
  data: Pi input; Pe input; Np input; RTi input; gamma input; dm input; t input; Ftg1 input; Ftg2 input; Ftg3 input; n output; eta output
function [n,eta]  = fcn(Pi, Pe, Np, RTi, gamma, dm, t , Ftg1, Ftg2, Ftg3)
Np = Np*1000;
N = Np*(1+Ftg2)/Ftg1;
k =  gamma/(gamma - 1);
theta = 1;
P0 = Pi*(theta+(1-theta)*(Pe/Pi)^(1/k))^(k);
ve = sqrt(2*k*RTi*(1-(Pe/P0)^(1/k)));
eta = 2*N*dm*Ftg3/(ve^2);

b1 = -1;
b2 = 4;
b3 = -eta;

coeff = [b1, b2, b3];
x_roots = roots(coeff);

phi = max(x_roots(x_roots > 0));

n = real(ve * phi/0.666);

if t <=1
    n =35500;
end

== matlab function rocket_sim/动力系统模块/煤油管路/MATLAB Function ==
  data: P_i input; dm_o output; dm_i input; m input; Fl1 input; P_e output; Fl2 input
function [dm_o, P_e] = pipe_dynamics(P_i,  dm_i,m, Fl1, Fl2)
    % 参数设置
    L = 0;    % 惯性流阻系数
    K = 0;    % 管路流阻系数
    C = 1;  % 流容系数
    f = 0.02;
    D = 0.6;
   LL = 10;
    A = (D/2)^2/4;
    rho = 820;
    delta_P = f*LL/(2*rho*1141*A*A*D)*dm_i^2;
  


    dm_o = dm_i*Fl1;

    P_e = (P_i -  L*dm_o/Fl1 - Fl2*K*m^2-delta_P)/C;

    
end
